simulink model "two_chamber_membrane_scaling"  (R2025b)
settings: Solver=VariableStepAuto  StartTime=0.0  StopTime=12000  RelTol=1e-3  AbsTol=1e-3
libraries: customization_lib x10, fl_lib x6, nesl_utility x6, simulink_extras x5
settings Model: Creator=degoede  LastModifiedBy=ndegoede
settings SolverCC: AutoScaleAbsTol=off
settings SimscapeCC: SimscapeLogType=all  SimscapeLogSimulationStatistics=on  SimscapeLogOpenViewer=on

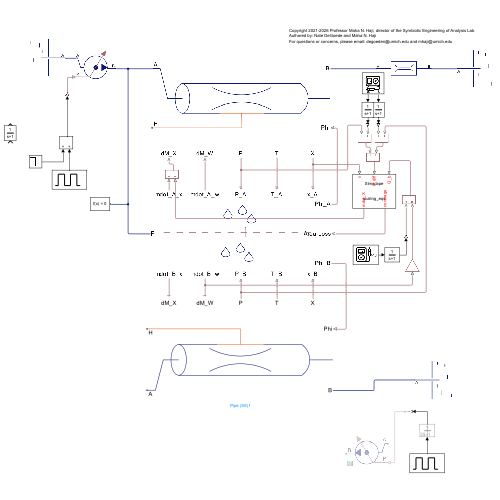
[thumbnail: Simulink's stored preview of the top-level diagram]
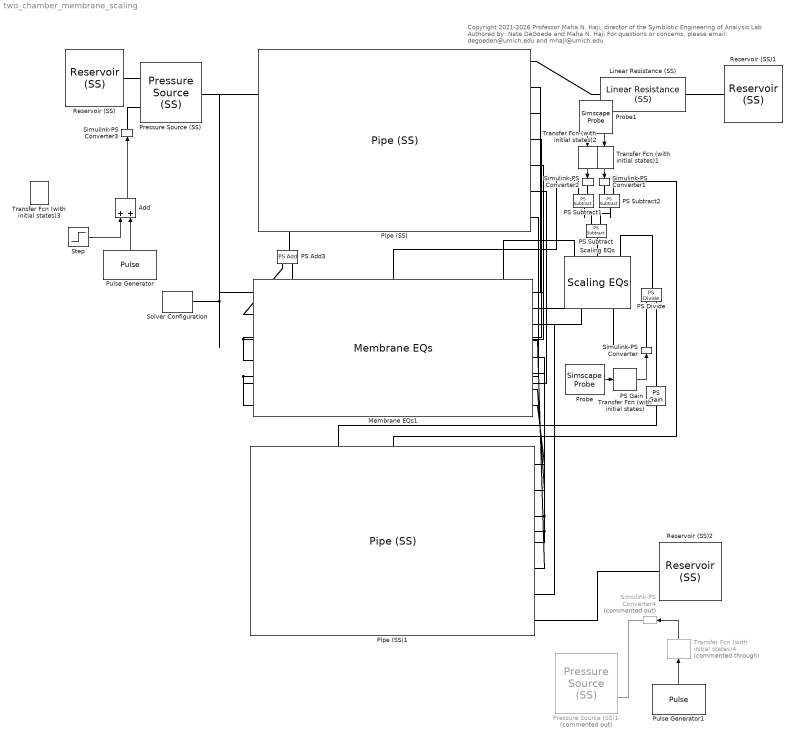
== system two_chamber_membrane_scaling ==
  note: Copyright 2021-2026 Professor Maha N. Haji, director of the Symbiotic Engineering of Analysis Lab
      | Authored by: Nate DeGoede and Maha N. Haji
      | For questions or concerns, please email: degoeden@umich.edu and mhaji@umich.edu
  Add : Sum
  Linear Resistance (SS) : customization_lib/solution/elements/Linear Resistance (SS)  R=64230000000 Pa*s/m^3  area=0.01 m^2
      settings: SourceProductName=Customization  InternalSimscapePortConfiguration="{\"Bottom\":[],\"Left\":[{\"id\":\"A\",\"label\":\"A\",\"type\":\"customization.solution.solution\"}],\"Right\":[{\"id\":\"B\",\"label\":\"B\",\"type\":\"customization.solution.solution\"}],\"Top\":[]}"
  Membrane EQs1 : customization_lib/membranes/Membrane EQs  A_w=4.269e-12 m^3/(N*s)  B_s=2.30e-8 m/s  A_m=1.2*0.4 m^2
      settings: SourceProductName=Customization  InternalSimscapePortConfiguration="{\"Bottom\":[{\"id\":\"mdot_B_x\",\"label\":\"mdot_B_x\",\"type\":\"output\"},{\"id\":\"mdot_B_w\",\"label\":\"mdot_B_w\",\"type\":\"output\"},{\"id\":\"P_B\",\"label\":\"P_B\",\"type\":\"input\"},{\"id\":\"T_B\",\"label\":\"T_B\",\"type\":\"input\"},{\"id\":\"x_B\",\"label\":\"x_B\",\"type\":\"input\"}],\"Left\":[{\"id\":\"F\",\"label\":\"F\",\"type\":\"customization.solution.solution\"}],\"Right\":[{\"id\":\"Phi_A\",\"label\":\"Phi_A\",\"type\":\"output\"},{\"id\":\"a_loss\",\"label\":\"Area Loss\",\"type\":\"input\"},{\"id\":\"Phi_B\",\"label\":\"Phi_B\",\"type\":\"output\"}],\"Top\":[{\"id\":\"mdot_A_x\",\"label\":\"mdot_A_x\",\"type\":\"output\"},{\"id\":\"mdot_A_w\",\"label\":\"mdot_A_w\",\"type\":\"output\"},{\"id\":\"P_A\",\"label\":\"P_A\",\"type\":\"input\"},{\"id\":\"T_A\",\"label\":\"T_A\",\"type\":\"input\"},{\"id\":\"x_A\",\"label\":\"x_A\",\"type\":\"input\"}]}"
  PS Add3 : fl_lib/Physical Signals/Functions/PS Add
  PS Divide : fl_lib/Physical Signals/Functions/PS Divide
  PS Gain : fl_lib/Physical Signals/Functions/PS Gain  gain=-1
  PS Subtract : fl_lib/Physical Signals/Functions/PS Subtract
  PS Subtract1 : fl_lib/Physical Signals/Functions/PS Subtract
  PS Subtract2 : fl_lib/Physical Signals/Functions/PS Subtract
  Pipe (SS) : customization_lib/solution/elements/Pipe (SS)  length=0.4 m  area=714 mm^2  Dh=0.7437 mm  length_add=0 m  roughness=1.5e-05 m  Re_lam=2000  Re_tur=4000  shape_factor=64  Nu_lam=3.66  dynamic_compressibility=true  inertia=false  p0=6 MPa  T0=293.15 K  x0=10.6 kg/m^3  mdot0=0 kg/s  m_measure=false  p_measure=true  t_measure=true  x_measure=true
      settings: SourceProductName=Customization  InternalSimscapePortConfiguration="{\"Bottom\":[{\"id\":\"dM_X\",\"label\":\"dM_X\",\"type\":\"input\"},{\"id\":\"dM_W\",\"label\":\"dM_W\",\"type\":\"input\"},{\"id\":\"P\",\"label\":\"P\",\"type\":\"output\"},{\"id\":\"T\",\"label\":\"T\",\"type\":\"output\"},{\"id\":\"X\",\"label\":\"X\",\"type\":\"output\"}],\"Left\":[{\"id\":\"A\",\"label\":\"A\",\"type\":\"customization.solution.solution\"},{\"id\":\"H\",\"label\":\"H\",\"type\":\"foundation.thermal.thermal\"}],\"Right\":[{\"id\":\"B\",\"label\":\"B\",\"type\":\"customization.solution.solution\"},{\"id\":\"Phi\",\"label\":\"Phi\",\"type\":\"input\"}],\"Top\":[]}"
  Pipe (SS)1 : customization_lib/solution/elements/Pipe (SS)  length=0.4 m  area=490.873852123405 mm^2  Dh=25 mm  length_add=0 m  roughness=1.5e-05 m  Re_lam=2000  Re_tur=4000  shape_factor=64  Nu_lam=3.66  dynamic_compressibility=true  inertia=false  p0=0.101 MPa  T0=293.15 K  x0=0 kg/m^3  mdot0=0 kg/s  m_measure=false  p_measure=true  t_measure=true  x_measure=true
      settings: SourceProductName=Customization  InternalSimscapePortConfiguration="{\"Bottom\":[{\"id\":\"dM_X\",\"label\":\"dM_X\",\"type\":\"input\"},{\"id\":\"dM_W\",\"label\":\"dM_W\",\"type\":\"input\"},{\"id\":\"P\",\"label\":\"P\",\"type\":\"output\"},{\"id\":\"T\",\"label\":\"T\",\"type\":\"output\"},{\"id\":\"X\",\"label\":\"X\",\"type\":\"output\"}],\"Left\":[{\"id\":\"A\",\"label\":\"A\",\"type\":\"customization.solution.solution\"},{\"id\":\"H\",\"label\":\"H\",\"type\":\"foundation.thermal.thermal\"}],\"Right\":[{\"id\":\"B\",\"label\":\"B\",\"type\":\"customization.solution.solution\"},{\"id\":\"Phi\",\"label\":\"Phi\",\"type\":\"input\"}],\"Top\":[]}"
  Pressure Source (SS) : customization_lib/solution/sources/Pressure Source (SS)  source_type=foundation.enum.constant_controlled.controlled  pressure_differential=0 MPa  power_spec=foundation.enum.power_spec.isentropic  area=0.01 m^2
      settings: SourceProductName=Customization  InternalSimscapePortConfiguration="{\"Bottom\":[],\"Left\":[{\"id\":\"A\",\"label\":\"A\",\"type\":\"customization.solution.solution\"},{\"id\":\"P\",\"label\":\"P\",\"type\":\"input\"}],\"Right\":[{\"id\":\"B\",\"label\":\"B\",\"type\":\"customization.solution.solution\"}],\"Top\":[]}"
  Pressure Source (SS)1 : customization_lib/solution/sources/Pressure Source (SS)  Commented=on  source_type=foundation.enum.constant_controlled.controlled  pressure_differential=0 MPa  power_spec=foundation.enum.power_spec.isentropic  area=0.01 m^2
      settings: SourceProductName=Customization  InternalSimscapePortConfiguration="{\"Bottom\":[],\"Left\":[{\"id\":\"A\",\"label\":\"A\",\"type\":\"customization.solution.solution\"},{\"id\":\"P\",\"label\":\"P\",\"type\":\"input\"}],\"Right\":[{\"id\":\"B\",\"label\":\"B\",\"type\":\"customization.solution.solution\"}],\"Top\":[]}"
  Probe : SimscapeProbe  BoundBlock=62  Variables="{\"rho_I\":{\"Probing\":\"ON\"}}"
  Probe1 : SimscapeProbe  BoundBlock=68  Variables="{\"pi_A\":{\"Probing\":\"ON\"},\"pi_B\":{\"Probing\":\"ON\"}}"
  Pulse Generator : DiscretePulseGenerator  PulseType=Time based  Amplitude=6  Period=6e3  PulseWidth=100 - 0.333333333333  PhaseDelay=50*60
  Pulse Generator1 : DiscretePulseGenerator  PulseType=Time based  Amplitude=10  Period=6e3  PulseWidth=0.333333333333  PhaseDelay=150*60
  Reservoir (SS) : customization_lib/solution/elements/Reservoir (SS)  pressure_spec=foundation.enum.pressure_spec.atmospheric  reservoir_pressure=6 MPa  reservoir_temperature=293.15 K  reservoir_concentration=10.6 kg/m^3  area=1 cm^2
      settings: SourceProductName=Customization  InternalSimscapePortConfiguration="{\"Bottom\":[],\"Left\":[{\"id\":\"A\",\"label\":\"A\",\"type\":\"customization.solution.solution\"}],\"Right\":[],\"Top\":[]}"
  Reservoir (SS)1 : customization_lib/solution/elements/Reservoir (SS)  pressure_spec=foundation.enum.pressure_spec.atmospheric  reservoir_pressure=0.101325 MPa  reservoir_temperature=293.15 K  reservoir_concentration=30 kg/m^3  area=27 mm^2
      settings: SourceProductName=Customization  InternalSimscapePortConfiguration="{\"Bottom\":[],\"Left\":[{\"id\":\"A\",\"label\":\"A\",\"type\":\"customization.solution.solution\"}],\"Right\":[],\"Top\":[]}"
  Reservoir (SS)2 : customization_lib/solution/elements/Reservoir (SS)  pressure_spec=foundation.enum.pressure_spec.atmospheric  reservoir_pressure=7 MPa  reservoir_temperature=293.15 K  reservoir_concentration=0 kg/m^3  area=1 cm^2
      settings: SourceProductName=Customization  InternalSimscapePortConfiguration="{\"Bottom\":[],\"Left\":[{\"id\":\"A\",\"label\":\"A\",\"type\":\"customization.solution.solution\"}],\"Right\":[],\"Top\":[]}"
  Scaling EQs : customization_lib/scaling/Scaling EQs  x_eq=5.89e-3 kg/m^3  K_G=22.6e-9 m/s  s=1  A_nucleation=1.777e-11 m^2  A_max=1.2*0.4 m^2  aspect_ratio=6.606e-3  scales_per_area=3e4 1/cm^2  F_detach=100 N  alpha=253 1/m  F_detach_buffer=1 N  scale_density=2711 kg/m^3  M_scale_specify=off  M_scale_priority=Low  M_scale=0 kg  M_scale_nominal_specify=off  M_scale_nominal_value=1  M_scale_nominal_unit=kg  Mdot_specify=off  Mdot_priority=None  Mdot=0 kg/s  Mdot_nominal_specify=off  Mdot_nominal_value=1  Mdot_nominal_unit=kg/s
      settings: SourceProductName=Customization  InternalSimscapePortConfiguration="{\"Bottom\":[],\"Left\":[{\"id\":\"x\",\"label\":\"x\",\"type\":\"input\"},{\"id\":\"P_diff\",\"label\":\"P_diff\",\"type\":\"input\"},{\"id\":\"Q_b\",\"label\":\"Q_b\",\"type\":\"input\"}],\"Right\":[{\"id\":\"mdot_x\",\"label\":\"mdot_X\",\"type\":\"output\"},{\"id\":\"coverage\",\"label\":\"coverage\",\"type\":\"output\"}],\"Top\":[]}"
  Simulink-PS Converter : nesl_utility/Simulink-PS Converter  PhysicalDomain=network_engine_domain  SubClassName=ps_input  LeftPortType=input  RightPortType=output  PseudoPeriodic=off  Frequencies=[]  NoiseDistribution=none  NoiseParameters=[]  Unit=kg/m^3  AffineConversion=off  FilteringAndDerivatives=provide  SimscapeFilterOrder=1  InputFilterTimeConstant=0.001  UdotUserProvided=0
  Simulink-PS Converter1 : nesl_utility/Simulink-PS Converter  PhysicalDomain=network_engine_domain  SubClassName=ps_input  LeftPortType=input  RightPortType=output  PseudoPeriodic=off  Frequencies=[]  NoiseDistribution=none  NoiseParameters=[]  Unit=Pa  AffineConversion=off  FilteringAndDerivatives=provide  SimscapeFilterOrder=1  InputFilterTimeConstant=0.001  UdotUserProvided=0
  Simulink-PS Converter2 : nesl_utility/Simulink-PS Converter  PhysicalDomain=network_engine_domain  SubClassName=ps_input  LeftPortType=input  RightPortType=output  PseudoPeriodic=off  Frequencies=[]  NoiseDistribution=none  NoiseParameters=[]  Unit=Pa  AffineConversion=off  FilteringAndDerivatives=provide  SimscapeFilterOrder=1  InputFilterTimeConstant=0.001  UdotUserProvided=0
  Simulink-PS Converter3 : nesl_utility/Simulink-PS Converter  PhysicalDomain=network_engine_domain  SubClassName=ps_input  LeftPortType=input  RightPortType=output  PseudoPeriodic=off  Frequencies=[]  NoiseDistribution=none  NoiseParameters=[]  Unit=MPa  AffineConversion=off  FilteringAndDerivatives=provide  SimscapeFilterOrder=1  InputFilterTimeConstant=0.001  UdotUserProvided=0
  Simulink-PS Converter4 : nesl_utility/Simulink-PS Converter  Commented=on  PhysicalDomain=network_engine_domain  SubClassName=ps_input  LeftPortType=input  RightPortType=output  PseudoPeriodic=off  Frequencies=[]  NoiseDistribution=none  NoiseParameters=[]  Unit=MPa  AffineConversion=off  FilteringAndDerivatives=provide  SimscapeFilterOrder=1  InputFilterTimeConstant=0.001  UdotUserProvided=0
  Solver Configuration : nesl_utility/Solver Configuration  PhysicalDomain=network_engine_domain  SubClassName=solver  LeftPortType=input  RightPortType=generic  Tones=[]  Harmonics=[]  SimulateNoise=off  Profile=off  UseLocalSampling=off  EnableSwitchedLinearOptims=on  FrequencyDomain=off  UseCCode=off  RelTol=0.001  AbsTol=0.001  MinStep=1e-09  ToWorkspace=off  RevertToSquareIcSolve=off  NumHomotopyIterations=100  PhasorMode=off  PhasorModeNumHarmonics=1  ConsistencySolver=NEWTON_XTOL_AFTER_FTOL  IndexReductionMethod=DerivativeReplacement  DoDC=off  ResidualTolerance=1e-09  ConsistencyTolSource=GLOBAL  ConsistencyAbsTol=0.001  ConsistencyRelTol=0.001  ConsistencyTolFactor=0.001  UseLocalSolver=off  LocalSolverChoice=NE_BACKWARD_EULER_ADVANCER  ResolveIndetEquations=on  FunctionEvalNumThread=1  LocalSolverSampleTime=0.001  DoFixedCost=off  MaxNonlinIter=3  MaxModeIter=2  ComputeImpulses=off  ImpulseIterations=2  LinearAlgebra=auto  LinearAlgebraNumThread=0  EquationFormulation=NE_TIME_EF  DelaysMemoryBudget=1024  AutomaticFiltering=off  FilteringTimeConstant=0.001  PartitionStorageMethod=AS_NEEDED  PartitionMemoryBudget=1024  PartitionMethod=ROBUST  MultibodyUseLocalSolver=off  MultibodyLocalSolverChoice=ODE1  MultibodyLocalSolverSampleTime=0.001
  Step : Step  Time=50*60  Before=6  After=0  SampleTime=0
  Transfer Fcn (with initial states) : simulink_extras/Additional Linear/Transfer Fcn (with initial states)  N=[1]  D="[1  1]"  X0=998.2
  Transfer Fcn (with initial states)1 : simulink_extras/Additional Linear/Transfer Fcn (with initial states)  N=[1]  D="[1  1]"  X0=0
  Transfer Fcn (with initial states)2 : simulink_extras/Additional Linear/Transfer Fcn (with initial states)  N=[1]  D="[1  1]"  X0=2.5e6
  Transfer Fcn (with initial states)3 : simulink_extras/Additional Linear/Transfer Fcn (with initial states)  N=[1]  D="[1  1]"  X0=6
  Transfer Fcn (with initial states)4 : simulink_extras/Additional Linear/Transfer Fcn (with initial states)  Commented=through  N=[1]  D="[1  1]"  X0=6
  wires:
  Probe/1 -> Transfer Fcn (with initial states)/1
  Transfer Fcn (with initial states)/1 -> Simulink-PS Converter/1
  Probe1/2 -> Transfer Fcn (with initial states)1/1
  Transfer Fcn (with initial states)1/1 -> Simulink-PS Converter1/1
  Probe1/1 -> Transfer Fcn (with initial states)2/1
  Transfer Fcn (with initial states)2/1 -> Simulink-PS Converter2/1
  Add/1 -> Simulink-PS Converter3/1
  Pulse Generator1/1 -> Transfer Fcn (with initial states)4/1
  Transfer Fcn (with initial states)4/1 -> Simulink-PS Converter4/1
  Pulse Generator/1 -> Add/2
  Step/1 -> Add/1
  connections:
  Solver Configuration/RConn1 -- Pipe (SS)/LConn1 -- Pressure Source (SS)/RConn1 -- Membrane EQs1/LConn1
  Linear Resistance (SS)/RConn1 -- Reservoir (SS)1/LConn1
  Membrane EQs1/RConn1 -- Pipe (SS)/RConn2
  Linear Resistance (SS)/LConn1 -- Pipe (SS)/RConn1
  Membrane EQs1/LConn6 -- Scaling EQs/LConn1 -- Pipe (SS)/RConn7
  Membrane EQs1/RConn3 -- Pipe (SS)1/RConn2
  Pipe (SS)1/RConn7 -- Membrane EQs1/RConn8
  Pipe (SS)1/RConn6 -- Membrane EQs1/RConn7
  Pipe (SS)1/RConn5 -- PS Subtract2/LConn1 -- Membrane EQs1/RConn6
  Pipe (SS)1/RConn4 -- PS Gain/LConn1 -- Membrane EQs1/RConn5
  Pipe (SS)1/RConn3 -- Membrane EQs1/RConn4
  Membrane EQs1/LConn2 -- PS Add3/LConn2
  Membrane EQs1/LConn3 -- Pipe (SS)/RConn4
  Membrane EQs1/LConn4 -- PS Subtract1/LConn1 -- Pipe (SS)/RConn5
  Membrane EQs1/LConn5 -- Pipe (SS)/RConn6
  Scaling EQs/RConn1 -- PS Add3/LConn1
  Pipe (SS)/RConn3 -- PS Add3/RConn1
  Scaling EQs/RConn2 -- Membrane EQs1/RConn2
  PS Subtract/RConn1 -- Scaling EQs/LConn2
  Simulink-PS Converter/RConn1 -- PS Divide/LConn2
  PS Gain/RConn1 -- PS Divide/LConn1
  PS Divide/RConn1 -- Scaling EQs/LConn3
  PS Subtract2/LConn2 -- Simulink-PS Converter1/RConn1
  PS Subtract1/LConn2 -- Simulink-PS Converter2/RConn1
  PS Subtract1/RConn1 -- PS Subtract/LConn1
  PS Subtract2/RConn1 -- PS Subtract/LConn2
  Reservoir (SS)/LConn1 -- Pressure Source (SS)/LConn1
  Simulink-PS Converter3/RConn1 -- Pressure Source (SS)/LConn2
  Simulink-PS Converter4/RConn1 -- Pressure Source (SS)1/LConn2
  Reservoir (SS)2/LConn1 -- Pipe (SS)1/RConn1
